simulink model "quad_control"  (R2026a)
settings: Solver=ode45  StopTime=20  MaxStep=0.01  RelTol=1e-6
PostLoadFcn:
  | if ~exist('konfiguracja', 'var') || ~strcmp(konfiguracja, 'LAB6'), run(fullfile(fileparts(get_param('quad_control', 'FileName')), 'parametry.m')); end
InitFcn:
  | if ~exist('konfiguracja', 'var') || ~strcmp(konfiguracja, 'LAB6'), run(fullfile(fileparts(get_param('quad_control', 'FileName')), 'parametry.m')); end
values from neighbouring files (symbols this model uses):
  CDxS = [0.0390 0.0455 0.0900]    [parametry.m]
  CQ = 0.00206    [parametry.m]
  CT = 0.0142    [parametry.m]
  d = 0.225    [parametry.m]    (also in run_lab6.m = squeeze(ts.Data))
  g = [0; 0; 9.81]    [parametry.m]    (also in run_lab6.m = t >= 30)
  Gust = [0 0 0]    [parametry.m]
  InitialPosition = [0 0 -10]    [parametry.m]
  m = 1.5    [parametry.m]
  R = 0.127    [parametry.m]    (also in run_lab6.m = struct())
  rho = 1.225    [parametry.m]
  t_gust = 20    [parametry.m]
  t_skok = 1    [parametry.m]
  tryb = 1    [parametry.m]
  v_xy = 0.5    [parametry.m]
  Wind = [0 0 0]    [parametry.m]
  Wmax = 1000    [parametry.m]
undefined symbols (not defined in the file or in its folder): Quadcopter
libraries: slpidlib x6, simulink x4
settings Model: Creator=felipekrystianek  LastModifiedBy=felipekrystianek

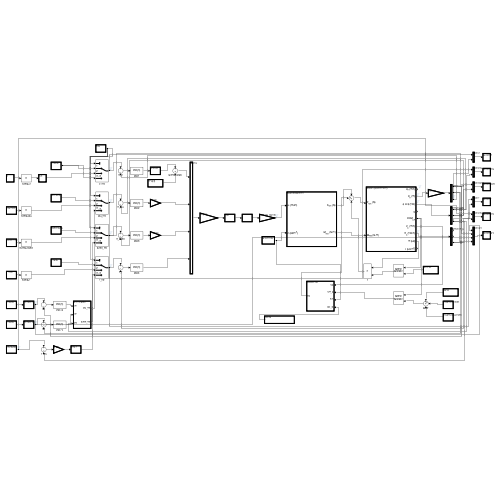
[thumbnail: Simulink's stored preview of the top-level diagram]
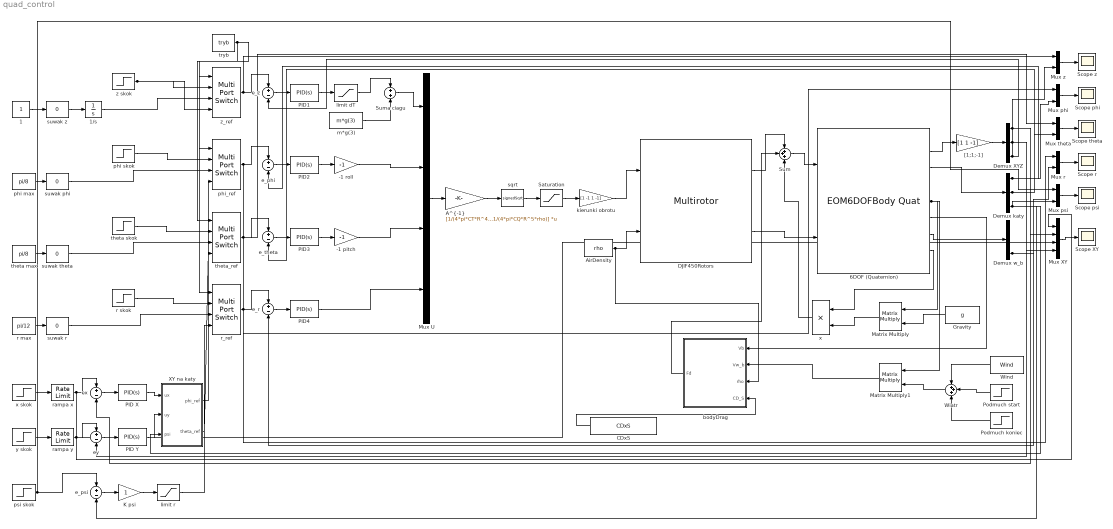
== system quad_control ==
  -1 pitch : Gain  Gain=-1
  -1 roll : Gain  Gain=-1
  1 : Constant
  1/s : Integrator  InitialCondition=-InitialPosition(3)
  6DOF (Quaternion) : EOM6DOFBodyQuat  xme_0=InitialPosition  mass_0=m  inertia=I  mass_flag=on
  "A^{-1}" : Gain  Gain=[1/(4*pi*CT*R^4*rho), 0, -1/(2*pi*CT*R^4*d*rho), -1/(4*pi*CQ*R^5*rho); 1/(4*pi*CT*R^4*rho), 1/(2*pi*CT*R^4*d*rho), 0, 1/(4*pi*CQ*R^5*rho); 1/(4*pi*CT*R^4*rho), 0, 1/(2*pi*CT*R^4*d*rho), -1/(4*pi*CQ*R^5*rho); 1/(4*pi*CT*R^4*rho), -1/(2*pi*CT*R^4*d*rho), 0, 1/(4*pi*CQ*R^5*rho)]  Multiplication=Matrix(K*u)
  AirDensity : Constant  Value=rho
  CDxS : Constant  Value=CDxS
  DJIF450Rotors : Multirotor  config=Quadcopter +  armLength=d  rotorHeight=H  CT=CT  CQ=CQ  radius=R
  Demux XYZ : Demux  Outputs=3
  Demux katy : Demux  Outputs=3
  Demux w_b : Demux  Outputs=3
  Gravity : Constant  Value=g
  K psi : Gain
  Matrix Multiply : Product  Multiplication=Matrix(*)
  Matrix Multiply1 : Product  Multiplication=Matrix(*)
  Mux U : Mux
  Mux XY : Mux
  Mux phi : Mux  Inputs=2
  Mux psi : Mux  Inputs=2
  Mux r : Mux  Inputs=2
  Mux theta : Mux  Inputs=2
  Mux z : Mux  Inputs=2
  PID X : slpidlib/PID Controller  Controller=PID  Form=Parallel  TimeDomain=Continuous-time  UseExternalTs=off  SampleTime=-1  IntegratorMethod=Forward Euler  FilterMethod=Forward Euler  ControllerParametersSource=internal  P=0.06  I=0.01  UseKiTs=off  D=0.3  UseExternalDerivativeSource=off  N=10  UseFilter=on  TunerSelectOption=Transfer Function Based (PID Tuner App)  InitialConditionSource=internal  InitialConditionForIntegrator=0  InitialConditionForFilter=0  DifferentiatorICPrevScaledInput=0  ExternalReset=none  TrackingMode=off  Kt=1  LimitOutput=off  SatLimitsSource=internal  UpperSaturationLimit=inf  LowerSaturationLimit=-inf  LinearizeAsGain=on  AntiWindupMode=none  Kb=1  LimitIntegrator=off  UpperIntegratorSaturationLimit=inf  LowerIntegratorSaturationLimit=-inf  POutMin=[]  POutMax=[]  IOutMin=[]  IOutMax=[]  DOutMin=[]  DOutMax=[]  NOutMin=[]  NOutMax=[]  SumOutMin=[]  SumOutMax=[]  SaturationOutMin=[]  SaturationOutMax=[]  PParamMin=[]  PParamMax=[]  IParamMin=[]  IParamMax=[]  DParamMin=[]  DParamMax=[]  NParamMin=[]  NParamMax=[]  KbParamMin=[]  KbParamMax=[]  KtParamMin=[]  KtParamMax=[]  KbOutMin=[]  KbOutMax=[]  KtOutMin=[]  KtOutMax=[]  IntegratorOutMin=[]  IntegratorOutMax=[]  FilterOutMin=[]  FilterOutMax=[]  SumI1OutMin=[]  SumI1OutMax=[]  SumI2OutMin=[]  SumI2OutMax=[]  SumI3OutMin=[]  SumI3OutMax=[]  SumI4OutMin=[]  SumI4OutMax=[]  SumDOutMin=[]  SumDOutMax=[]  DifferentiatorOutMin=[]  DifferentiatorOutMax=[]  FilterDiffOutCoefMin=[]  FilterDiffOutCoefMax=[]  ReciprocalOutMin=[]  ReciprocalOutMax=[]  SumDenOutMin=[]  SumDenOutMax=[]  SumNumOutMin=[]  SumNumOutMax=[]  DivideOutMin=[]  DivideOutMax=[]  UdiffTsProdOutMin=[]  UdiffTsProdOutMax=[]  NTsProdOutMin=[]  NTsProdOutMax=[]  UintegralTsProdOutMin=[]  UintegralTsProdOutMax=[]  UngainTsProdOutMin=[]  UngainTsProdOutMax=[]  ClampingZeroOutDataTypeStr=Inherit: Inherit via back propagation  ClampingZeroOutMin=[]  ClampingZeroOutMax=[]  FilterDenConstantOutDataTypeStr=Inherit: Inherit via back propagation  FilterDenConstantOutMin=[]  FilterDenConstantOutMax=[]  PCopyOutDataTypeStr=Inherit: Inherit via back propagation  PCopyOutMin=[]  PCopyOutMax=[]  NCopyOutDataTypeStr=Inherit: Inherit via back propagation  NCopyOutMin=[]  NCopyOutMax=[]  IntegratorContinuousStateAttributes=''  IntegratorStateMustResolveToSignalObject=off  IntegratorRTWStateStorageClass=Auto  FilterContinuousStateAttributes=''  FilterStateMustResolveToSignalObject=off  FilterRTWStateStorageClass=Auto  ParallelPVariant=InternalParameters  IdealPVariant=Disabled  IVariant=InternalParameters  DVariant=InternalParameters  IntegratorVariant=Continuous  SatVariant=Disabled  AWVariant=Passthrough  PCopyVariant=Disabled  TRVariant=Disabled  FdbkBlocksVariant=Forward  IdealPFdbkVariant=Disabled  SatFdbkVariant=Disabled  DerivativeFilterVariant=ContFilter  NVariant=InternalParameters  NCopyVariant=Disabled  FilterICVariant=InternalICsFilter  IntegratorICVariant=InternalICs  ExternalResetVariant=Disabled  TRSumVariant=Passthrough  SumFdbkVariant=Disabled  SumVariant=Sum_PID  TsampFilterVariant=InternalTs  TsampNgainVariant=Passthrough  TsampIntegralVariant=Disabled_SignalSpec  ExternalSaturationOutDataTypeStr=Inherit: Same as second input  DerivativeSourceVariant=ErrorSignal  PreIntVariant=InternalPreInt
  PID Y : slpidlib/PID Controller  Controller=PID  Form=Parallel  TimeDomain=Continuous-time  UseExternalTs=off  SampleTime=-1  IntegratorMethod=Forward Euler  FilterMethod=Forward Euler  ControllerParametersSource=internal  P=0.06  I=0.01  UseKiTs=off  D=0.3  UseExternalDerivativeSource=off  N=10  UseFilter=on  TunerSelectOption=Transfer Function Based (PID Tuner App)  InitialConditionSource=internal  InitialConditionForIntegrator=0  InitialConditionForFilter=0  DifferentiatorICPrevScaledInput=0  ExternalReset=none  TrackingMode=off  Kt=1  LimitOutput=off  SatLimitsSource=internal  UpperSaturationLimit=inf  LowerSaturationLimit=-inf  LinearizeAsGain=on  AntiWindupMode=none  Kb=1  LimitIntegrator=off  UpperIntegratorSaturationLimit=inf  LowerIntegratorSaturationLimit=-inf  POutMin=[]  POutMax=[]  IOutMin=[]  IOutMax=[]  DOutMin=[]  DOutMax=[]  NOutMin=[]  NOutMax=[]  SumOutMin=[]  SumOutMax=[]  SaturationOutMin=[]  SaturationOutMax=[]  PParamMin=[]  PParamMax=[]  IParamMin=[]  IParamMax=[]  DParamMin=[]  DParamMax=[]  NParamMin=[]  NParamMax=[]  KbParamMin=[]  KbParamMax=[]  KtParamMin=[]  KtParamMax=[]  KbOutMin=[]  KbOutMax=[]  KtOutMin=[]  KtOutMax=[]  IntegratorOutMin=[]  IntegratorOutMax=[]  FilterOutMin=[]  FilterOutMax=[]  SumI1OutMin=[]  SumI1OutMax=[]  SumI2OutMin=[]  SumI2OutMax=[]  SumI3OutMin=[]  SumI3OutMax=[]  SumI4OutMin=[]  SumI4OutMax=[]  SumDOutMin=[]  SumDOutMax=[]  DifferentiatorOutMin=[]  DifferentiatorOutMax=[]  FilterDiffOutCoefMin=[]  FilterDiffOutCoefMax=[]  ReciprocalOutMin=[]  ReciprocalOutMax=[]  SumDenOutMin=[]  SumDenOutMax=[]  SumNumOutMin=[]  SumNumOutMax=[]  DivideOutMin=[]  DivideOutMax=[]  UdiffTsProdOutMin=[]  UdiffTsProdOutMax=[]  NTsProdOutMin=[]  NTsProdOutMax=[]  UintegralTsProdOutMin=[]  UintegralTsProdOutMax=[]  UngainTsProdOutMin=[]  UngainTsProdOutMax=[]  ClampingZeroOutDataTypeStr=Inherit: Inherit via back propagation  ClampingZeroOutMin=[]  ClampingZeroOutMax=[]  FilterDenConstantOutDataTypeStr=Inherit: Inherit via back propagation  FilterDenConstantOutMin=[]  FilterDenConstantOutMax=[]  PCopyOutDataTypeStr=Inherit: Inherit via back propagation  PCopyOutMin=[]  PCopyOutMax=[]  NCopyOutDataTypeStr=Inherit: Inherit via back propagation  NCopyOutMin=[]  NCopyOutMax=[]  IntegratorContinuousStateAttributes=''  IntegratorStateMustResolveToSignalObject=off  IntegratorRTWStateStorageClass=Auto  FilterContinuousStateAttributes=''  FilterStateMustResolveToSignalObject=off  FilterRTWStateStorageClass=Auto  ParallelPVariant=InternalParameters  IdealPVariant=Disabled  IVariant=InternalParameters  DVariant=InternalParameters  IntegratorVariant=Continuous  SatVariant=Disabled  AWVariant=Passthrough  PCopyVariant=Disabled  TRVariant=Disabled  FdbkBlocksVariant=Forward  IdealPFdbkVariant=Disabled  SatFdbkVariant=Disabled  DerivativeFilterVariant=ContFilter  NVariant=InternalParameters  NCopyVariant=Disabled  FilterICVariant=InternalICsFilter  IntegratorICVariant=InternalICs  ExternalResetVariant=Disabled  TRSumVariant=Passthrough  SumFdbkVariant=Disabled  SumVariant=Sum_PID  TsampFilterVariant=InternalTs  TsampNgainVariant=Passthrough  TsampIntegralVariant=Disabled_SignalSpec  ExternalSaturationOutDataTypeStr=Inherit: Same as second input  DerivativeSourceVariant=ErrorSignal  PreIntVariant=InternalPreInt
  PID1 : slpidlib/PID Controller  Controller=PID  Form=Parallel  TimeDomain=Continuous-time  UseExternalTs=off  SampleTime=-1  IntegratorMethod=Forward Euler  FilterMethod=Forward Euler  ControllerParametersSource=internal  P=20  I=0.001  UseKiTs=off  D=30  UseExternalDerivativeSource=off  N=10  UseFilter=on  TunerSelectOption=Transfer Function Based (PID Tuner App)  InitialConditionSource=internal  InitialConditionForIntegrator=0  InitialConditionForFilter=0  DifferentiatorICPrevScaledInput=0  ExternalReset=none  TrackingMode=off  Kt=1  LimitOutput=off  SatLimitsSource=internal  UpperSaturationLimit=inf  LowerSaturationLimit=-inf  LinearizeAsGain=on  AntiWindupMode=none  Kb=1  LimitIntegrator=off  UpperIntegratorSaturationLimit=inf  LowerIntegratorSaturationLimit=-inf  POutMin=[]  POutMax=[]  IOutMin=[]  IOutMax=[]  DOutMin=[]  DOutMax=[]  NOutMin=[]  NOutMax=[]  SumOutMin=[]  SumOutMax=[]  SaturationOutMin=[]  SaturationOutMax=[]  PParamMin=[]  PParamMax=[]  IParamMin=[]  IParamMax=[]  DParamMin=[]  DParamMax=[]  NParamMin=[]  NParamMax=[]  KbParamMin=[]  KbParamMax=[]  KtParamMin=[]  KtParamMax=[]  KbOutMin=[]  KbOutMax=[]  KtOutMin=[]  KtOutMax=[]  IntegratorOutMin=[]  IntegratorOutMax=[]  FilterOutMin=[]  FilterOutMax=[]  SumI1OutMin=[]  SumI1OutMax=[]  SumI2OutMin=[]  SumI2OutMax=[]  SumI3OutMin=[]  SumI3OutMax=[]  SumI4OutMin=[]  SumI4OutMax=[]  SumDOutMin=[]  SumDOutMax=[]  DifferentiatorOutMin=[]  DifferentiatorOutMax=[]  FilterDiffOutCoefMin=[]  FilterDiffOutCoefMax=[]  ReciprocalOutMin=[]  ReciprocalOutMax=[]  SumDenOutMin=[]  SumDenOutMax=[]  SumNumOutMin=[]  SumNumOutMax=[]  DivideOutMin=[]  DivideOutMax=[]  UdiffTsProdOutMin=[]  UdiffTsProdOutMax=[]  NTsProdOutMin=[]  NTsProdOutMax=[]  UintegralTsProdOutMin=[]  UintegralTsProdOutMax=[]  UngainTsProdOutMin=[]  UngainTsProdOutMax=[]  ClampingZeroOutDataTypeStr=Inherit: Inherit via back propagation  ClampingZeroOutMin=[]  ClampingZeroOutMax=[]  FilterDenConstantOutDataTypeStr=Inherit: Inherit via back propagation  FilterDenConstantOutMin=[]  FilterDenConstantOutMax=[]  PCopyOutDataTypeStr=Inherit: Inherit via back propagation  PCopyOutMin=[]  PCopyOutMax=[]  NCopyOutDataTypeStr=Inherit: Inherit via back propagation  NCopyOutMin=[]  NCopyOutMax=[]  IntegratorContinuousStateAttributes=''  IntegratorStateMustResolveToSignalObject=off  IntegratorRTWStateStorageClass=Auto  FilterContinuousStateAttributes=''  FilterStateMustResolveToSignalObject=off  FilterRTWStateStorageClass=Auto  ParallelPVariant=InternalParameters  IdealPVariant=Disabled  IVariant=InternalParameters  DVariant=InternalParameters  IntegratorVariant=Continuous  SatVariant=Disabled  AWVariant=Passthrough  PCopyVariant=Disabled  TRVariant=Disabled  FdbkBlocksVariant=Forward  IdealPFdbkVariant=Disabled  SatFdbkVariant=Disabled  DerivativeFilterVariant=ContFilter  NVariant=InternalParameters  NCopyVariant=Disabled  FilterICVariant=InternalICsFilter  IntegratorICVariant=InternalICs  ExternalResetVariant=Disabled  TRSumVariant=Passthrough  SumFdbkVariant=Disabled  SumVariant=Sum_PID  TsampFilterVariant=InternalTs  TsampNgainVariant=Passthrough  TsampIntegralVariant=Disabled_SignalSpec  ExternalSaturationOutDataTypeStr=Inherit: Same as second input  DerivativeSourceVariant=ErrorSignal  PreIntVariant=InternalPreInt
  PID2 : slpidlib/PID Controller  Controller=PID  Form=Parallel  TimeDomain=Continuous-time  UseExternalTs=off  SampleTime=-1  IntegratorMethod=Forward Euler  FilterMethod=Forward Euler  ControllerParametersSource=internal  P=0.00042  I=2.87e-6  UseKiTs=off  D=0.011  UseExternalDerivativeSource=off  N=10  UseFilter=on  TunerSelectOption=Transfer Function Based (PID Tuner App)  InitialConditionSource=internal  InitialConditionForIntegrator=0  InitialConditionForFilter=0  DifferentiatorICPrevScaledInput=0  ExternalReset=none  TrackingMode=off  Kt=1  LimitOutput=off  SatLimitsSource=internal  UpperSaturationLimit=inf  LowerSaturationLimit=-inf  LinearizeAsGain=on  AntiWindupMode=none  Kb=1  LimitIntegrator=off  UpperIntegratorSaturationLimit=inf  LowerIntegratorSaturationLimit=-inf  POutMin=[]  POutMax=[]  IOutMin=[]  IOutMax=[]  DOutMin=[]  DOutMax=[]  NOutMin=[]  NOutMax=[]  SumOutMin=[]  SumOutMax=[]  SaturationOutMin=[]  SaturationOutMax=[]  PParamMin=[]  PParamMax=[]  IParamMin=[]  IParamMax=[]  DParamMin=[]  DParamMax=[]  NParamMin=[]  NParamMax=[]  KbParamMin=[]  KbParamMax=[]  KtParamMin=[]  KtParamMax=[]  KbOutMin=[]  KbOutMax=[]  KtOutMin=[]  KtOutMax=[]  IntegratorOutMin=[]  IntegratorOutMax=[]  FilterOutMin=[]  FilterOutMax=[]  SumI1OutMin=[]  SumI1OutMax=[]  SumI2OutMin=[]  SumI2OutMax=[]  SumI3OutMin=[]  SumI3OutMax=[]  SumI4OutMin=[]  SumI4OutMax=[]  SumDOutMin=[]  SumDOutMax=[]  DifferentiatorOutMin=[]  DifferentiatorOutMax=[]  FilterDiffOutCoefMin=[]  FilterDiffOutCoefMax=[]  ReciprocalOutMin=[]  ReciprocalOutMax=[]  SumDenOutMin=[]  SumDenOutMax=[]  SumNumOutMin=[]  SumNumOutMax=[]  DivideOutMin=[]  DivideOutMax=[]  UdiffTsProdOutMin=[]  UdiffTsProdOutMax=[]  NTsProdOutMin=[]  NTsProdOutMax=[]  UintegralTsProdOutMin=[]  UintegralTsProdOutMax=[]  UngainTsProdOutMin=[]  UngainTsProdOutMax=[]  ClampingZeroOutDataTypeStr=Inherit: Inherit via back propagation  ClampingZeroOutMin=[]  ClampingZeroOutMax=[]  FilterDenConstantOutDataTypeStr=Inherit: Inherit via back propagation  FilterDenConstantOutMin=[]  FilterDenConstantOutMax=[]  PCopyOutDataTypeStr=Inherit: Inherit via back propagation  PCopyOutMin=[]  PCopyOutMax=[]  NCopyOutDataTypeStr=Inherit: Inherit via back propagation  NCopyOutMin=[]  NCopyOutMax=[]  IntegratorContinuousStateAttributes=''  IntegratorStateMustResolveToSignalObject=off  IntegratorRTWStateStorageClass=Auto  FilterContinuousStateAttributes=''  FilterStateMustResolveToSignalObject=off  FilterRTWStateStorageClass=Auto  ParallelPVariant=InternalParameters  IdealPVariant=Disabled  IVariant=InternalParameters  DVariant=InternalParameters  IntegratorVariant=Continuous  SatVariant=Disabled  AWVariant=Passthrough  PCopyVariant=Disabled  TRVariant=Disabled  FdbkBlocksVariant=Forward  IdealPFdbkVariant=Disabled  SatFdbkVariant=Disabled  DerivativeFilterVariant=ContFilter  NVariant=InternalParameters  NCopyVariant=Disabled  FilterICVariant=InternalICsFilter  IntegratorICVariant=InternalICs  ExternalResetVariant=Disabled  TRSumVariant=Passthrough  SumFdbkVariant=Disabled  SumVariant=Sum_PID  TsampFilterVariant=InternalTs  TsampNgainVariant=Passthrough  TsampIntegralVariant=Disabled_SignalSpec  ExternalSaturationOutDataTypeStr=Inherit: Same as second input  DerivativeSourceVariant=ErrorSignal  PreIntVariant=InternalPreInt
  PID3 : slpidlib/PID Controller  Controller=PID  Form=Parallel  TimeDomain=Continuous-time  UseExternalTs=off  SampleTime=-1  IntegratorMethod=Forward Euler  FilterMethod=Forward Euler  ControllerParametersSource=internal  P=0.0038  I=9.97e-5  UseKiTs=off  D=0.026  UseExternalDerivativeSource=off  N=10  UseFilter=on  TunerSelectOption=Transfer Function Based (PID Tuner App)  InitialConditionSource=internal  InitialConditionForIntegrator=0  InitialConditionForFilter=0  DifferentiatorICPrevScaledInput=0  ExternalReset=none  TrackingMode=off  Kt=1  LimitOutput=off  SatLimitsSource=internal  UpperSaturationLimit=inf  LowerSaturationLimit=-inf  LinearizeAsGain=on  AntiWindupMode=none  Kb=1  LimitIntegrator=off  UpperIntegratorSaturationLimit=inf  LowerIntegratorSaturationLimit=-inf  POutMin=[]  POutMax=[]  IOutMin=[]  IOutMax=[]  DOutMin=[]  DOutMax=[]  NOutMin=[]  NOutMax=[]  SumOutMin=[]  SumOutMax=[]  SaturationOutMin=[]  SaturationOutMax=[]  PParamMin=[]  PParamMax=[]  IParamMin=[]  IParamMax=[]  DParamMin=[]  DParamMax=[]  NParamMin=[]  NParamMax=[]  KbParamMin=[]  KbParamMax=[]  KtParamMin=[]  KtParamMax=[]  KbOutMin=[]  KbOutMax=[]  KtOutMin=[]  KtOutMax=[]  IntegratorOutMin=[]  IntegratorOutMax=[]  FilterOutMin=[]  FilterOutMax=[]  SumI1OutMin=[]  SumI1OutMax=[]  SumI2OutMin=[]  SumI2OutMax=[]  SumI3OutMin=[]  SumI3OutMax=[]  SumI4OutMin=[]  SumI4OutMax=[]  SumDOutMin=[]  SumDOutMax=[]  DifferentiatorOutMin=[]  DifferentiatorOutMax=[]  FilterDiffOutCoefMin=[]  FilterDiffOutCoefMax=[]  ReciprocalOutMin=[]  ReciprocalOutMax=[]  SumDenOutMin=[]  SumDenOutMax=[]  SumNumOutMin=[]  SumNumOutMax=[]  DivideOutMin=[]  DivideOutMax=[]  UdiffTsProdOutMin=[]  UdiffTsProdOutMax=[]  NTsProdOutMin=[]  NTsProdOutMax=[]  UintegralTsProdOutMin=[]  UintegralTsProdOutMax=[]  UngainTsProdOutMin=[]  UngainTsProdOutMax=[]  ClampingZeroOutDataTypeStr=Inherit: Inherit via back propagation  ClampingZeroOutMin=[]  ClampingZeroOutMax=[]  FilterDenConstantOutDataTypeStr=Inherit: Inherit via back propagation  FilterDenConstantOutMin=[]  FilterDenConstantOutMax=[]  PCopyOutDataTypeStr=Inherit: Inherit via back propagation  PCopyOutMin=[]  PCopyOutMax=[]  NCopyOutDataTypeStr=Inherit: Inherit via back propagation  NCopyOutMin=[]  NCopyOutMax=[]  IntegratorContinuousStateAttributes=''  IntegratorStateMustResolveToSignalObject=off  IntegratorRTWStateStorageClass=Auto  FilterContinuousStateAttributes=''  FilterStateMustResolveToSignalObject=off  FilterRTWStateStorageClass=Auto  ParallelPVariant=InternalParameters  IdealPVariant=Disabled  IVariant=InternalParameters  DVariant=InternalParameters  IntegratorVariant=Continuous  SatVariant=Disabled  AWVariant=Passthrough  PCopyVariant=Disabled  TRVariant=Disabled  FdbkBlocksVariant=Forward  IdealPFdbkVariant=Disabled  SatFdbkVariant=Disabled  DerivativeFilterVariant=ContFilter  NVariant=InternalParameters  NCopyVariant=Disabled  FilterICVariant=InternalICsFilter  IntegratorICVariant=InternalICs  ExternalResetVariant=Disabled  TRSumVariant=Passthrough  SumFdbkVariant=Disabled  SumVariant=Sum_PID  TsampFilterVariant=InternalTs  TsampNgainVariant=Passthrough  TsampIntegralVariant=Disabled_SignalSpec  ExternalSaturationOutDataTypeStr=Inherit: Same as second input  DerivativeSourceVariant=ErrorSignal  PreIntVariant=InternalPreInt
  PID4 : slpidlib/PID Controller  Controller=PID  Form=Parallel  TimeDomain=Continuous-time  UseExternalTs=off  SampleTime=-1  IntegratorMethod=Forward Euler  FilterMethod=Forward Euler  ControllerParametersSource=internal  P=0.020  I=0.0093  UseKiTs=off  D=0.0014  UseExternalDerivativeSource=off  N=10  UseFilter=on  TunerSelectOption=Transfer Function Based (PID Tuner App)  InitialConditionSource=internal  InitialConditionForIntegrator=0  InitialConditionForFilter=0  DifferentiatorICPrevScaledInput=0  ExternalReset=none  TrackingMode=off  Kt=1  LimitOutput=off  SatLimitsSource=internal  UpperSaturationLimit=inf  LowerSaturationLimit=-inf  LinearizeAsGain=on  AntiWindupMode=none  Kb=1  LimitIntegrator=off  UpperIntegratorSaturationLimit=inf  LowerIntegratorSaturationLimit=-inf  POutMin=[]  POutMax=[]  IOutMin=[]  IOutMax=[]  DOutMin=[]  DOutMax=[]  NOutMin=[]  NOutMax=[]  SumOutMin=[]  SumOutMax=[]  SaturationOutMin=[]  SaturationOutMax=[]  PParamMin=[]  PParamMax=[]  IParamMin=[]  IParamMax=[]  DParamMin=[]  DParamMax=[]  NParamMin=[]  NParamMax=[]  KbParamMin=[]  KbParamMax=[]  KtParamMin=[]  KtParamMax=[]  KbOutMin=[]  KbOutMax=[]  KtOutMin=[]  KtOutMax=[]  IntegratorOutMin=[]  IntegratorOutMax=[]  FilterOutMin=[]  FilterOutMax=[]  SumI1OutMin=[]  SumI1OutMax=[]  SumI2OutMin=[]  SumI2OutMax=[]  SumI3OutMin=[]  SumI3OutMax=[]  SumI4OutMin=[]  SumI4OutMax=[]  SumDOutMin=[]  SumDOutMax=[]  DifferentiatorOutMin=[]  DifferentiatorOutMax=[]  FilterDiffOutCoefMin=[]  FilterDiffOutCoefMax=[]  ReciprocalOutMin=[]  ReciprocalOutMax=[]  SumDenOutMin=[]  SumDenOutMax=[]  SumNumOutMin=[]  SumNumOutMax=[]  DivideOutMin=[]  DivideOutMax=[]  UdiffTsProdOutMin=[]  UdiffTsProdOutMax=[]  NTsProdOutMin=[]  NTsProdOutMax=[]  UintegralTsProdOutMin=[]  UintegralTsProdOutMax=[]  UngainTsProdOutMin=[]  UngainTsProdOutMax=[]  ClampingZeroOutDataTypeStr=Inherit: Inherit via back propagation  ClampingZeroOutMin=[]  ClampingZeroOutMax=[]  FilterDenConstantOutDataTypeStr=Inherit: Inherit via back propagation  FilterDenConstantOutMin=[]  FilterDenConstantOutMax=[]  PCopyOutDataTypeStr=Inherit: Inherit via back propagation  PCopyOutMin=[]  PCopyOutMax=[]  NCopyOutDataTypeStr=Inherit: Inherit via back propagation  NCopyOutMin=[]  NCopyOutMax=[]  IntegratorContinuousStateAttributes=''  IntegratorStateMustResolveToSignalObject=off  IntegratorRTWStateStorageClass=Auto  FilterContinuousStateAttributes=''  FilterStateMustResolveToSignalObject=off  FilterRTWStateStorageClass=Auto  ParallelPVariant=InternalParameters  IdealPVariant=Disabled  IVariant=InternalParameters  DVariant=InternalParameters  IntegratorVariant=Continuous  SatVariant=Disabled  AWVariant=Passthrough  PCopyVariant=Disabled  TRVariant=Disabled  FdbkBlocksVariant=Forward  IdealPFdbkVariant=Disabled  SatFdbkVariant=Disabled  DerivativeFilterVariant=ContFilter  NVariant=InternalParameters  NCopyVariant=Disabled  FilterICVariant=InternalICsFilter  IntegratorICVariant=InternalICs  ExternalResetVariant=Disabled  TRSumVariant=Passthrough  SumFdbkVariant=Disabled  SumVariant=Sum_PID  TsampFilterVariant=InternalTs  TsampNgainVariant=Passthrough  TsampIntegralVariant=Disabled_SignalSpec  ExternalSaturationOutDataTypeStr=Inherit: Same as second input  DerivativeSourceVariant=ErrorSignal  PreIntVariant=InternalPreInt
  Podmuch koniec : Step  Time=t_gust + 2  InitialValue=[0 0 0]  FinalValue=-Gust  SampleTime=0
  Podmuch start : Step  Time=t_gust  InitialValue=[0 0 0]  FinalValue=Gust  SampleTime=0
  Saturation : Saturate  UpperLimit=Wmax  LowerLimit=0
  Scope XY : Scope
      settings: Title=XY  YLabel=x, y [m]
  Scope phi : Scope
      settings: Title=phi  YLabel=\phi [rad]
  Scope psi : Scope
      settings: Title=psi  YLabel=\psi [rad]
  Scope r : Scope
      settings: Title=r  YLabel=r [rad/s]
  Scope theta : Scope
      settings: Title=theta  YLabel=\theta [rad]
  Scope z : Scope
      settings: Title=z  YLabel=z [m]
  Sum : Sum  Inputs=+++
  Suma ciagu : Sum
  Wiatr : Sum  Inputs=+++
  Wind : Constant  Value=Wind
  XY na katy : MATLAB Function  TreatAsAtomicUnit=on
  "[1;1;-1]" : Gain  Gain=[1 1 -1]
  bodyDrag : MATLAB Function  TreatAsAtomicUnit=on
  e_phi : Sum  Inputs=+-
  e_psi : Sum  Inputs=+-
  e_r : Sum  Inputs=+-
  e_theta : Sum  Inputs=+-
  e_z : Sum  Inputs=+-
  ex : Sum  Inputs=+-
  ey : Sum  Inputs=+-
  kierunki obrotu : Gain  Gain=[1 -1 1 -1]
  limit dT : Saturate  UpperLimit=0.5*m*g(3)  LowerLimit=-0.5*m*g(3)
  limit r : Saturate  UpperLimit=pi/12  LowerLimit=-pi/12
  m*g(3) : Constant  Value=m*g(3)
  phi max : Constant  Value=pi/8
  phi skok : Step  Time=t_skok  FinalValue=phi_cel  SampleTime=0
  phi_ref : MultiPortSwitch  SaturateOnIntegerOverflow=off  InputSameDT=off
  psi skok : Step  Time=t_skok  FinalValue=psi_cel  SampleTime=0
  r max : Constant  Value=pi/12
  r skok : Step  Time=t_skok  FinalValue=r_cel  SampleTime=0
  r_ref : MultiPortSwitch  SaturateOnIntegerOverflow=off  InputSameDT=off
  rampa x : RateLimiter  RisingSlewLimit=v_xy  FallingSlewLimit=-v_xy  SampleTimeMode=inherited
  rampa y : RateLimiter  RisingSlewLimit=v_xy  FallingSlewLimit=-v_xy  SampleTimeMode=inherited
  sqrt : Sqrt  Operator=signedSqrt
  suwak phi : simulink/Math Operations/Slider Gain  gain=0  low=-1  high=1
  suwak r : simulink/Math Operations/Slider Gain  gain=0  low=-1  high=1
  suwak theta : simulink/Math Operations/Slider Gain  gain=0  low=-1  high=1
  suwak z : simulink/Math Operations/Slider Gain  gain=0  low=-1  high=1
  theta max : Constant  Value=pi/8
  theta skok : Step  Time=t_skok  FinalValue=theta_cel  SampleTime=0
  theta_ref : MultiPortSwitch  SaturateOnIntegerOverflow=off  InputSameDT=off
  tryb : Constant  Value=tryb
  x : Product
  x skok : Step  Time=t_skok  FinalValue=x_cel  SampleTime=0
  y skok : Step  Time=t_skok  FinalValue=y_cel  SampleTime=0
  z skok : Step  Time=t_skok  InitialValue=-InitialPosition(3)  FinalValue=z_cel  SampleTime=0
  z_ref : MultiPortSwitch  SaturateOnIntegerOverflow=off  InputSameDT=off
  wires:
  AirDensity/1 -> DJIF450Rotors/2, bodyDrag/3(rho)
  DJIF450Rotors/1 -> Sum/1
  DJIF450Rotors/2 -> 6DOF (Quaternion)/2
  Sum/1 -> 6DOF (Quaternion)/1
  6DOF (Quaternion)/5 -> Matrix Multiply/1, Matrix Multiply1/1
  Gravity/1 -> Matrix Multiply/2
  6DOF (Quaternion)/8 -> x/1
  Matrix Multiply/1 -> x/2
  x/1 -> Sum/3
  Wind/1 -> Wiatr/1
  Podmuch start/1 -> Wiatr/2
  Podmuch koniec/1 -> Wiatr/3
  Wiatr/1 -> Matrix Multiply1/2
  6DOF (Quaternion)/6 -> bodyDrag/1(Vb)
  Matrix Multiply1/1 -> bodyDrag/2(Vw_b)
  CDxS/1 -> bodyDrag/4(CD_S)
  bodyDrag/1(Fd) -> Sum/2
  6DOF (Quaternion)/2 -> "[1;1;-1]"/1
  "[1;1;-1]"/1 -> Demux XYZ/1
  6DOF (Quaternion)/3 -> Demux katy/1
  6DOF (Quaternion)/7 -> Demux w_b/1
  1/1 -> suwak z/1
  suwak z/1 -> 1/s/1
  phi max/1 -> suwak phi/1
  theta max/1 -> suwak theta/1
  r max/1 -> suwak r/1
  tryb/1 -> z_ref/1, r_ref/1, phi_ref/1, theta_ref/1
  z skok/1 -> z_ref/2, z_ref/4
  1/s/1 -> z_ref/3
  r skok/1 -> r_ref/2
  suwak r/1 -> r_ref/3
  limit r/1 -> r_ref/4
  psi skok/1 -> e_psi/1, Mux psi/1
  Demux katy/3 -> e_psi/2, XY na katy/3(psi), Mux psi/2
  e_psi/1 -> K psi/1
  K psi/1 -> limit r/1
  phi skok/1 -> phi_ref/2
  suwak phi/1 -> phi_ref/3
  XY na katy/1(phi_ref) -> phi_ref/4
  theta skok/1 -> theta_ref/2
  suwak theta/1 -> theta_ref/3
  XY na katy/2(theta_ref) -> theta_ref/4
  x skok/1 -> rampa x/1
  rampa x/1 -> ex/1, Mux XY/1
  Demux XYZ/1 -> ex/2, Mux XY/2
  ex/1 -> PID X/1
  y skok/1 -> rampa y/1
  rampa y/1 -> ey/1, Mux XY/3
  Demux XYZ/2 -> ey/2, Mux XY/4
  ey/1 -> PID Y/1
  PID X/1 -> XY na katy/1(ux)
  PID Y/1 -> XY na katy/2(uy)
  z_ref/1 -> e_z/1, Mux z/1
  Demux XYZ/3 -> e_z/2, Mux z/2
  phi_ref/1 -> e_phi/1, Mux phi/1
  Demux katy/1 -> e_phi/2, Mux phi/2
  theta_ref/1 -> e_theta/1, Mux theta/1
  Demux katy/2 -> e_theta/2, Mux theta/2
  r_ref/1 -> e_r/1, Mux r/1
  Demux w_b/3 -> e_r/2, Mux r/2
  e_z/1 -> PID1/1
  e_phi/1 -> PID2/1
  e_theta/1 -> PID3/1
  e_r/1 -> PID4/1
  PID1/1 -> limit dT/1
  limit dT/1 -> Suma ciagu/1
  m*g(3)/1 -> Suma ciagu/2
  Suma ciagu/1 -> Mux U/1
  PID2/1 -> -1 roll/1
  -1 roll/1 -> Mux U/2
  PID3/1 -> -1 pitch/1
  -1 pitch/1 -> Mux U/3
  PID4/1 -> Mux U/4
  Mux U/1 -> "A^{-1}"/1
  "A^{-1}"/1 -> sqrt/1
  sqrt/1 -> Saturation/1
  Saturation/1 -> kierunki obrotu/1
  kierunki obrotu/1 -> DJIF450Rotors/1
  Mux z/1 -> Scope z/1
  Mux phi/1 -> Scope phi/1
  Mux theta/1 -> Scope theta/1
  Mux r/1 -> Scope r/1
  Mux psi/1 -> Scope psi/1
  Mux XY/1 -> Scope XY/1

== matlab function quad_control/XY na katy ==
  data: ux input; phi_ref output; uy input; psi input; theta_ref output
function [phi_ref, theta_ref] = xy_na_katy(ux, uy, psi) %#codegen
% Zamienia wyjscia regulatorow X, Y (uklad ziemski) na zadane katy roll i pitch.
% Najpierw obrot o kat yaw do ukladu BSP, potem: zeby leciec do przodu (+x) BSP pochyla nos w dol
% (theta < 0), a zeby leciec w prawo (+y) przechyla sie w prawo (phi > 0).
kat_max = pi/8;                          % ograniczenie przechylenia
ub = cos(psi)*ux + sin(psi)*uy;          % do przodu w ukladzie BSP
vb = -sin(psi)*ux + cos(psi)*uy;         % w prawo w ukladzie BSP
theta_ref = min(max(-ub, -kat_max), kat_max);
phi_ref = min(max(vb, -kat_max), kat_max);
end

== matlab function quad_control/bodyDrag ==
  data: Vb input; Fd output; Vw_b input; rho input; CD_S input
function Fd = bodyDrag(Vb, Vw_b, rho, CD_S) %#codegen
% Sila oporu aerodynamicznego w ukladzie zwiazanym z BSP (jak na slajdzie 50 wykladu)
% Vb, Vw_b: [3x1] m/s; rho: kg/m^3; CD_S: [3x1] = [Cd_x*Sx; Cd_y*Sy; Cd_z*Sz] m^2
Vrel = Vb(:) - Vw_b(:);
Fdx = -0.5*rho*CD_S(1)*abs(Vrel(1))*Vrel(1);
Fdy = -0.5*rho*CD_S(2)*abs(Vrel(2))*Vrel(2);
Fdz = -0.5*rho*CD_S(3)*abs(Vrel(3))*Vrel(3);
Fd = [Fdx; Fdy; Fdz];
end
